simulink model "part1_pendulum_linearization"  (R2024b)
settings: Solver=ode45  StartTime=0.0  StopTime=2  MaxStep=0.005  RelTol=1e-8  AbsTol=1e-10
model workspace (MAT data in the model file):
  g = 9.81
  k = 0.05
  l = 0.5
  m = 0.2
  omega0 = 0
  theta0 = 0.1
settings Model: Creator=matiasgarcia  LastModifiedBy=matiasgarcia
settings DataIOCC: SaveOutput=off  SignalLogging=off  SaveTime=off

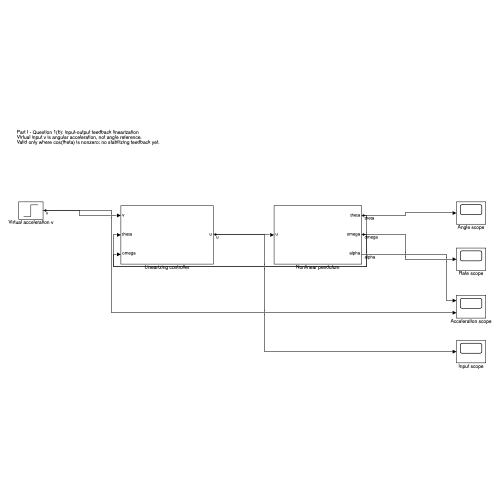
[thumbnail: Simulink's stored preview of the top-level diagram]
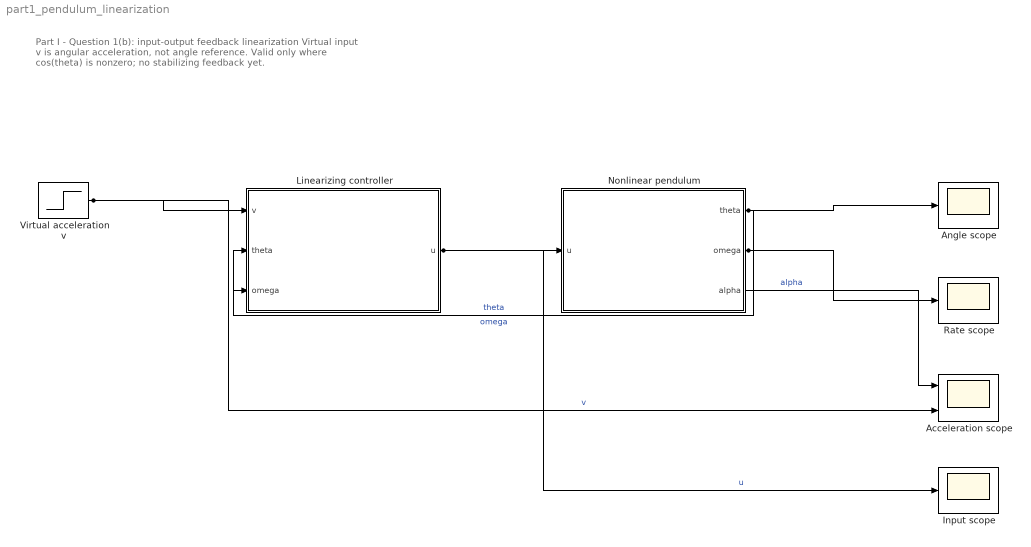
== system part1_pendulum_linearization ==
  note: Part I - Question 1(b): input-output feedback linearization
      | Virtual input v is angular acceleration, not angle reference.
      | Valid only where cos(theta) is nonzero; no stabilizing feedback yet.
  Acceleration scope : Scope  NumInputPorts=2
  Angle scope : Scope
  Input scope : Scope
  Linearizing controller : Subsystem
  Nonlinear pendulum : Subsystem
  Rate scope : Scope
  Virtual acceleration v : Step  Time=0.2  After=0.2  SampleTime=0
  wires:
  Virtual acceleration v/1 -> Linearizing controller/1(v), Acceleration scope/2  "v"
  Nonlinear pendulum/1(theta) -> Linearizing controller/2(theta), Angle scope/1  "theta"
  Nonlinear pendulum/2(omega) -> Linearizing controller/3(omega), Rate scope/1  "omega"
  Linearizing controller/1(u) -> Nonlinear pendulum/1(u), Input scope/1  "u"
  Nonlinear pendulum/3(alpha) -> Acceleration scope/1  "alpha"

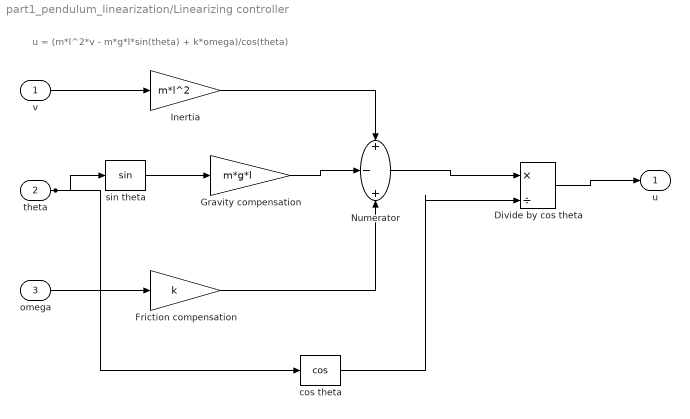
== system part1_pendulum_linearization/Linearizing controller ==
  note: u = (m*l^2*v - m*g*l*sin(theta) + k*omega)/cos(theta)
  v : Inport
  theta : Inport  Port=2
  omega : Inport  Port=3
  Divide by cos theta : Product  Inputs=*/
  Friction compensation : Gain  Gain=k
  Gravity compensation : Gain  Gain=m*g*l
  Inertia : Gain  Gain=m*l^2
  Numerator : Sum  Inputs=+-+
  cos theta : Trigonometry  Operator=cos
  sin theta : Trigonometry
  u : Outport
  wires:
  v/1 -> Inertia/1
  theta/1 -> sin theta/1, cos theta/1
  sin theta/1 -> Gravity compensation/1
  omega/1 -> Friction compensation/1
  Inertia/1 -> Numerator/1
  Gravity compensation/1 -> Numerator/2
  Friction compensation/1 -> Numerator/3
  Numerator/1 -> Divide by cos theta/1
  cos theta/1 -> Divide by cos theta/2
  Divide by cos theta/1 -> u/1

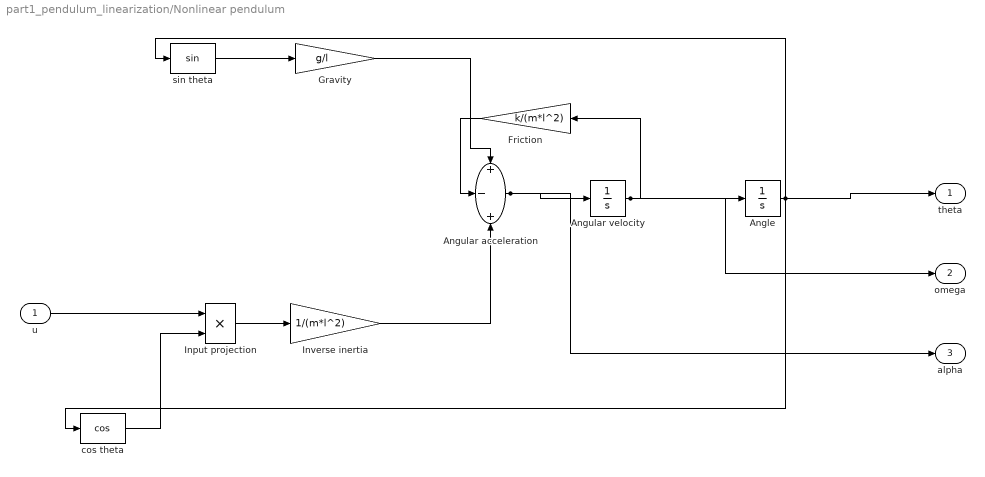
== system part1_pendulum_linearization/Nonlinear pendulum ==
  u : Inport
  Angle : Integrator  InitialCondition=theta0
  Angular acceleration : Sum  Inputs=+-+
  Angular velocity : Integrator  InitialCondition=omega0
  Friction : Gain  Gain=k/(m*l^2)
  Gravity : Gain  Gain=g/l
  Input projection : Product
  Inverse inertia : Gain  Gain=1/(m*l^2)
  cos theta : Trigonometry  Operator=cos
  sin theta : Trigonometry
  theta : Outport
  omega : Outport  Port=2
  alpha : Outport  Port=3
  wires:
  u/1 -> Input projection/1
  cos theta/1 -> Input projection/2
  Input projection/1 -> Inverse inertia/1
  Inverse inertia/1 -> Angular acceleration/3
  sin theta/1 -> Gravity/1
  Gravity/1 -> Angular acceleration/1
  Angular velocity/1 -> Friction/1, Angle/1, omega/1
  Friction/1 -> Angular acceleration/2
  Angular acceleration/1 -> Angular velocity/1, alpha/1
  Angle/1 -> sin theta/1, cos theta/1, theta/1
